simulink model "untitled"  (R2013a)
settings: Solver=ode45  StartTime=0.0  StopTime=10.0  RelTol=1e-3
values from neighbouring files (symbols this model uses):
  RA = 0.001    [MC.m]    (also in Model2.m; XX1.m = params.RA; XX2.m = params.RA; XX3.m = params.RA)
  RM = 0.005    [MC.m]    (also in Model2.m; XX1.m = params.RM; XX2.m = params.RM; XX3.m = params.RM)
undefined symbols (not defined in the file or in its folder): c, dc
settings Model: Creator=Mojtaba  LastModifiedBy=Mojtaba

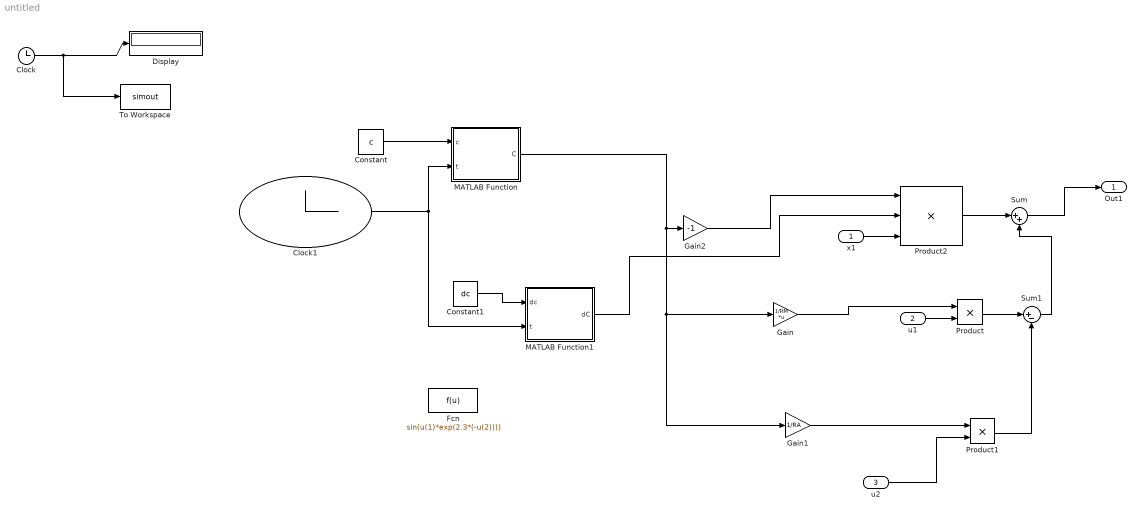
== system untitled ==
  x1 : Inport
  u1 : Inport  Port=2
  u2 : Inport  Port=3
  Clock : Clock
  Clock1 : Clock
  Constant : Constant  Value=c
  Constant1 : Constant  Value=dc
  Display : Display
  Fcn : Fcn  Expr=sin(u(1)*exp(2.3*(-u(2))))
  Gain : Gain  Gain=1/RM  Multiplication=Matrix(K*u) (u vector)
  Gain1 : Gain  Gain=1/RA
  Gain2 : Gain  Gain=-1
  MATLAB Function : MATLAB Function  TreatAsAtomicUnit=on
  MATLAB Function1 : MATLAB Function  TreatAsAtomicUnit=on
  Product : Product
  Product1 : Product
  Product2 : Product  Inputs=3
  Sum : Sum  Inputs=|++
  Sum1 : Sum  Inputs=|+-
  To Workspace : ToWorkspace  VariableName=simout  SampleTime=-1  SaveFormat=Timeseries
  Out1 : Outport
  wires:
  Clock/1 -> To Workspace/1, Display/1
  u2/1 -> Product1/2
  u1/1 -> Product/2
  Product1/1 -> Sum1/2
  Product/1 -> Sum1/1
  Sum1/1 -> Sum/2
  Sum/1 -> Out1/1
  Gain/1 -> Product/1
  Gain1/1 -> Product1/1
  Gain2/1 -> Product2/1
  x1/1 -> Product2/3
  Product2/1 -> Sum/1
  MATLAB Function1/1(dC) -> Product2/2
  MATLAB Function/1(C) -> Gain/1, Gain1/1, Gain2/1
  Clock1/1 -> MATLAB Function/2(t), MATLAB Function1/2(t)
  Constant/1 -> MATLAB Function/1(c)
  Constant1/1 -> MATLAB Function1/1(dc)

== matlab function untitled/MATLAB Function1 ==
  data: dc input; t input; dC output
function dC = fcn(dc,t)
dC =dc(t);
% Rs=1;
% RM=0.005;
% RA=0.001;
% Rc=0.0398;
% CR=4.4;
% Cs=1.33;
% CA=0.08;
% Ls=0.0005;
% Emax=2;
% Emin=0.06;
% Tmax=10; 
% HR=1;
% % Tn=(t/Tmax);
% % En= 1.55*(((Tn/0.7)^1.9)/((1+(Tn/0.7)^1.9)))*(1/(1+(Tn/1.17)^21.9));
% En= 1.55*((((t/Tmax)/0.7)^1.9)/((1+((t/Tmax)/0.7)^1.9)))*(1/(1+((t/Tmax)/1.17)^21.9));
% E=(Emax-Emin)*En+Emin;
% C=1/E;
% dc= ((589*(Emax - Emin)*((10*Tn)/7)^(14/5))/(140*(((10*Tn)/7)^(19/10) + 1)^2*(((100*Tn)/117)^(219/10) + 1)) - (589*(Emax - Emin)*((10*Tn)/7)^(9/10))/(140*(((10*Tn)/7)^(19/10) + 1)*(((100*Tn)/117)^(219/10) + 1)) + (2263*(Emax - Emin)*((10*Tn)/7)^(19/10)*((100*Tn)/117)^(209/10))/(78*(((10*Tn)/7)^(19/10) + 1)*(((100*Tn)/117)^(219/10) + 1)^2))/(Emin + (31*(Emax - Emin)*((10*Tn)/7)^(19/10))/(20*(((10*Tn)/7)^(19/10) + 1)*(((100*Tn)/117)^(219/10) + 1)))^2;
% dc= ((589*(Emax - Emin)*((10*(t/Tmax))/7)^(14/5))/(140*(((10*(t/Tmax))/7)^(19/10) + 1)^2*(((100*(t/Tmax))/117)^(219/10) + 1)) - (589*(Emax - Emin)*((10*(t/Tmax))/7)^(9/10))/(140*(((10*(t/Tmax))/7)^(19/10) + 1)*(((100*(t/Tmax))/117)^(219/10) + 1)) + (2263*(Emax - Emin)*((10*(t/Tmax))/7)^(19/10)*((100*(t/Tmax))/117)^(209/10))/(78*(((10*(t/Tmax))/7)^(19/10) + 1)*(((100*(t/Tmax))/117)^(219/10) + 1)^2))/(Emin + (31*(Emax - Emin)*((10*(t/Tmax))/7)^(19/10))/(20*(((10*(t/Tmax))/7)^(19/10) + 1)*(((100*(t/Tmax))/117)^(219/10) + 1)))^2;
% dC=dc;
end

== matlab function untitled/MATLAB Function ==
  data: c input; t input; C output
function C = fcn(c,t)
C=c(t);
% Rs=1;
% RM=0.005;
% RA=0.001;
% Rc=0.0398;
% CR=4.4;
% Cs=1.33;
% CA=0.08;
% Ls=0.0005;
% Emax=2;
% Emin=0.06;
% Tmax=10; 
% HR=1;

% Tn=(t/Tmax);
% En= 1.55*(((Tn/0.7)^1.9)/((1+(Tn/0.7)^1.9)))*(1/(1+(Tn/1.17)^21.9));
% En=1.55*((((t/Tmax)/0.7)^1.9)/((1+((t/Tmax)/0.7)^1.9)))*(1/(1+((t/Tmax)/1.17)^21.9));
% E=(Emax-Emin)*En+Emin;
% C=E;
% % dc= ((589*(Emax - Emin)*((10*Tn)/7)^(14/5))/(140*(((10*Tn)/7)^(19/10) + 1)^2*(((100*Tn)/117)^(219/10) + 1)) - (589*(Emax - Emin)*((10*Tn)/7)^(9/10))/(140*(((10*Tn)/7)^(19/10) + 1)*(((100*Tn)/117)^(219/10) + 1)) + (2263*(Emax - Emin)*((10*Tn)/7)^(19/10)*((100*Tn)/117)^(209/10))/(78*(((10*Tn)/7)^(19/10) + 1)*(((100*Tn)/117)^(219/10) + 1)^2))/(Emin + (31*(Emax - Emin)*((10*Tn)/7)^(19/10))/(20*(((10*Tn)/7)^(19/10) + 1)*(((100*Tn)/117)^(219/10) + 1)))^2;
% dc= ((589*(Emax - Emin)*((10*(t/Tmax))/7)^(14/5))/(140*(((10*(t/Tmax))/7)^(19/10) + 1)^2*(((100*(t/Tmax))/117)^(219/10) + 1)) - (589*(Emax - Emin)*((10*(t/Tmax))/7)^(9/10))/(140*(((10*(t/Tmax))/7)^(19/10) + 1)*(((100*(t/Tmax))/117)^(219/10) + 1)) + (2263*(Emax - Emin)*((10*(t/Tmax))/7)^(19/10)*((100*(t/Tmax))/117)^(209/10))/(78*(((10*(t/Tmax))/7)^(19/10) + 1)*(((100*(t/Tmax))/117)^(219/10) + 1)^2))/(Emin + (31*(Emax - Emin)*((10*(t/Tmax))/7)^(19/10))/(20*(((10*(t/Tmax))/7)^(19/10) + 1)*(((100*(t/Tmax))/117)^(219/10) + 1)))^2;
% dC=dc;
end
